simulink subsystem "complementaryFilter"  (R2026a)
settings: Solver=VariableStepAuto
values from neighbouring files (symbols this model uses):
  navComp = 0.995    [navParams.sldd]
  navControl = 1    [navParams.sldd]
undefined symbols (not defined in the file or in its folder): flightMode
libraries: simulink x3, vrlib x1, sharedutil x1
settings Model: Creator=maxhu  LastModifiedBy=maxhu

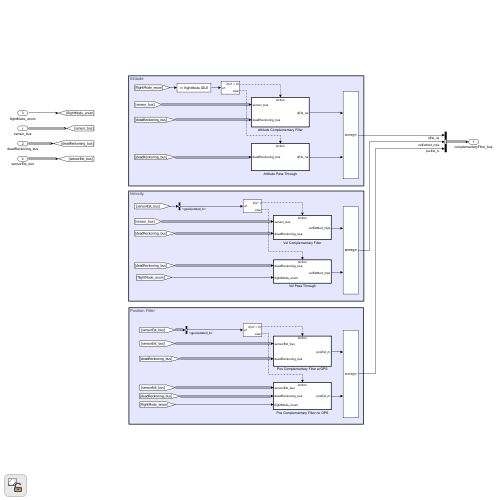
[thumbnail: Simulink's stored preview of the top-level diagram]
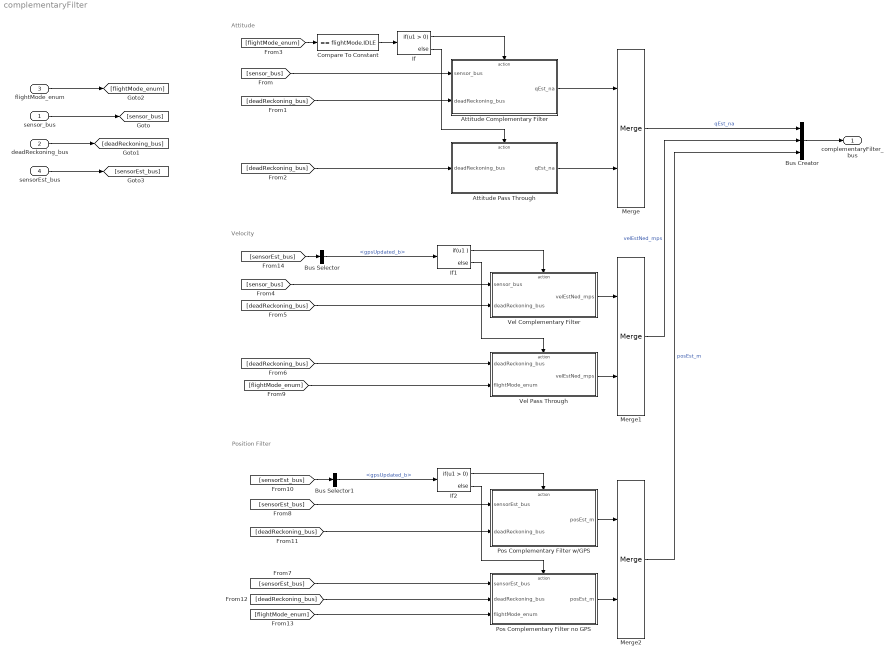
== system complementaryFilter ==
  note: Position Filter
  note: Attitude
  note: Velocity
  sensor_bus : Inport
  deadReckoning_bus : Inport  Port=2
  flightMode_enum : Inport  Port=3
  sensorEst_bus : Inport  Port=4
  Attitude Complementary Filter : Subsystem  TreatAsAtomicUnit=on
  Attitude Pass Through : Subsystem  TreatAsAtomicUnit=on
  Bus Creator : BusCreator  Inputs=3
  Bus Selector : BusSelector  OutputSignals=gpsUpdated_b
  Bus Selector1 : BusSelector  OutputSignals=gpsUpdated_b
  Compare To Constant : simulink/Logic and Bit Operations/Compare To Constant  relop===  const=flightMode.IDLE  OutDataTypeStr=boolean
  If : If
  If1 : If  IfExpression=u1
  If2 : If
  Merge : Merge
  Merge1 : Merge
  Merge2 : Merge
  Pos Complementary Filter no GPS : Subsystem  TreatAsAtomicUnit=on
  Pos Complementary Filter w/GPS : Subsystem  TreatAsAtomicUnit=on
  Vel Complementary Filter : Subsystem  TreatAsAtomicUnit=on
  Vel Pass Through : Subsystem  TreatAsAtomicUnit=on
  complementaryFilter_bus : Outport
  wires:
  Merge/1 -> Bus Creator/1  "qEst_na"
  Bus Creator/1 -> complementaryFilter_bus/1
  Compare To Constant/1 -> If/1
  If/1 -> Attitude Complementary Filter/Action
  If/2 -> Attitude Pass Through/Action
  Attitude Complementary Filter/1(qEst_na) -> Merge/1
  Attitude Pass Through/1(qEst_na) -> Merge/2
  [sensor_bus] -> Attitude Complementary Filter/1(sensor_bus)
  [deadReckoning_bus] -> Attitude Complementary Filter/2(deadReckoning_bus)
  [deadReckoning_bus] -> Attitude Pass Through/1(deadReckoning_bus)
  [flightMode_enum] -> Compare To Constant/1
  sensor_bus/1 -> [sensor_bus]
  deadReckoning_bus/1 -> [deadReckoning_bus]
  flightMode_enum/1 -> [flightMode_enum]
  Merge2/1 -> Bus Creator/3  "posEst_m"
  sensorEst_bus/1 -> [sensorEst_bus]
  If2/2 -> Pos Complementary Filter no GPS/Action
  Pos Complementary Filter no GPS/1(posEst_m) -> Merge2/2
  Pos Complementary Filter w/GPS/1(posEst_m) -> Merge2/1
  Bus Selector1/1 -> If2/1  "<gpsUpdated_b>"
  If2/1 -> Pos Complementary Filter w/GPS/Action
  [deadReckoning_bus] -> Pos Complementary Filter w/GPS/2(deadReckoning_bus)
  [deadReckoning_bus] -> Pos Complementary Filter no GPS/2(deadReckoning_bus)
  [sensorEst_bus] -> Pos Complementary Filter no GPS/1(sensorEst_bus)
  [sensorEst_bus] -> Pos Complementary Filter w/GPS/1(sensorEst_bus)
  [flightMode_enum] -> Pos Complementary Filter no GPS/3(flightMode_enum)
  If1/2 -> Vel Pass Through/Action
  Vel Complementary Filter/1(velEstNed_mps) -> Merge1/1
  [deadReckoning_bus] -> Vel Pass Through/1(deadReckoning_bus)
  Bus Selector/1 -> If1/1  "<gpsUpdated_b>"
  [flightMode_enum] -> Vel Pass Through/2(flightMode_enum)
  If1/1 -> Vel Complementary Filter/Action
  Vel Pass Through/1(velEstNed_mps) -> Merge1/2
  [sensor_bus] -> Vel Complementary Filter/1(sensor_bus)
  [deadReckoning_bus] -> Vel Complementary Filter/2(deadReckoning_bus)
  Merge1/1 -> Bus Creator/2  "velEstNed_mps"
  [sensorEst_bus] -> Bus Selector/1
  [sensorEst_bus] -> Bus Selector1/1

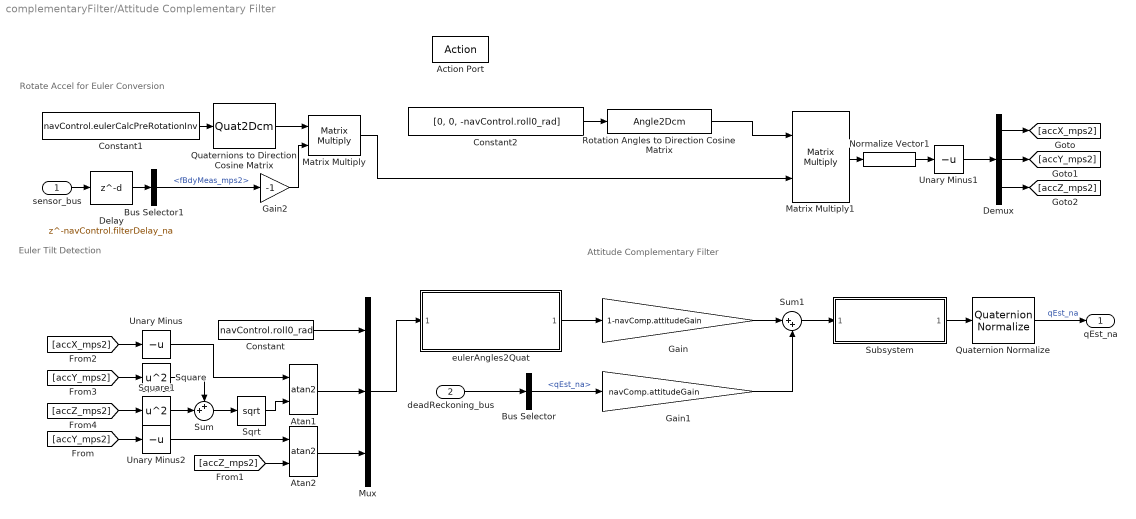
== system complementaryFilter/Attitude Complementary Filter ==
  note: Rotate Accel for Euler Conversion
  note: Euler Tilt Detection
  note: Attitude Complementary Filter
  sensor_bus : Inport
  deadReckoning_bus : Inport  Port=2
  Action Port : ActionPort
  Atan1 : Trigonometry  Operator=atan2
  Atan2 : Trigonometry  Operator=atan2
  Bus Selector : BusSelector  OutputSignals=qEst_na
  Bus Selector1 : BusSelector  OutputSignals=fBdyMeas_mps2
  Constant : Constant  Value=navControl.roll0_rad
  Constant1 : Constant  Value=navControl.eulerCalcPreRotationInv
  Constant2 : Constant  Value=[0, 0, -navControl.roll0_rad]
  Delay : Delay  DelayLength=navControl.filterDelay_na
  Demux : Demux  Outputs=3
  Gain : Gain  Gain=1-navComp.attitudeGain
  Gain1 : Gain  Gain=navComp.attitudeGain
  Gain2 : Gain  Gain=-1
  Matrix Multiply : Product  Multiplication=Matrix(*)
  Matrix Multiply1 : Product  Multiplication=Matrix(*)
  Mux : Mux  Inputs=3
  Normalize Vector1 : vrlib/Utilities/Normalize Vector  maxzero=1e-6
  Quaternion Normalize : sharedutil/Quaternion Normalize  aMode=aMode
  Quaternions to Direction Cosine Matrix : Quat2Dcm
  Rotation Angles to Direction Cosine Matrix : Angle2Dcm  rotationOrder=XYZ
      settings: AttributesFormatString=Rotation Order: %<rotationOrder>
  Sqrt : Sqrt
  Square : Math  Operator=square
  Square1 : Math  Operator=square
  Subsystem : Subsystem  ReferencedSubsystem=removeQuatZero
  Sum : Sum  Inputs=++|
  Sum1 : Sum  Inputs=|++
  Unary Minus : UnaryMinus
  Unary Minus1 : UnaryMinus
  Unary Minus2 : UnaryMinus
  eulerAngles2Quat : Subsystem  ReferencedSubsystem=eulerAngles2Quat
  qEst_na : Outport
  wires:
  Constant2/1 -> Rotation Angles to Direction Cosine Matrix/1
  Rotation Angles to Direction Cosine Matrix/1 -> Matrix Multiply1/1
  Constant/1 -> Mux/1
  Matrix Multiply1/1 -> Normalize Vector1/1
  Matrix Multiply/1 -> Matrix Multiply1/2
  Unary Minus2/1 -> Atan2/1
  Atan2/1 -> Mux/3
  Atan1/1 -> Mux/2
  Unary Minus1/1 -> Demux/1
  Normalize Vector1/1 -> Unary Minus1/1
  Unary Minus/1 -> Atan1/1
  Sqrt/1 -> Atan1/2
  [accY_mps2] -> Unary Minus2/1
  [accZ_mps2] -> Atan2/2
  Gain/1 -> Sum1/1
  [accY_mps2] -> Square/1
  Gain1/1 -> Sum1/2
  Square/1 -> Sum/1
  Sum/1 -> Sqrt/1
  eulerAngles2Quat/1 -> Gain/1
  Demux/1 -> [accX_mps2]
  Square1/1 -> Sum/2
  Demux/2 -> [accY_mps2]
  Demux/3 -> [accZ_mps2]
  [accX_mps2] -> Unary Minus/1
  [accZ_mps2] -> Square1/1
  deadReckoning_bus/1 -> Bus Selector/1
  Bus Selector/1 -> Gain1/1  "<qEst_na>"
  Gain2/1 -> Matrix Multiply/2
  sensor_bus/1 -> Delay/1
  Bus Selector1/1 -> Gain2/1  "<fBdyMeas_mps2>"
  Delay/1 -> Bus Selector1/1
  Quaternions to Direction Cosine Matrix/1 -> Matrix Multiply/1
  Constant1/1 -> Quaternions to Direction Cosine Matrix/1
  Mux/1 -> eulerAngles2Quat/1
  Quaternion Normalize/1 -> qEst_na/1  "qEst_na"
  Subsystem/1 -> Quaternion Normalize/1
  Sum1/1 -> Subsystem/1

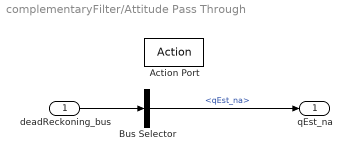
== system complementaryFilter/Attitude Pass Through ==
  deadReckoning_bus : Inport
  Action Port : ActionPort
  Bus Selector : BusSelector  OutputSignals=qEst_na
  qEst_na : Outport
  wires:
  Bus Selector/1 -> qEst_na/1  "<qEst_na>"
  deadReckoning_bus/1 -> Bus Selector/1

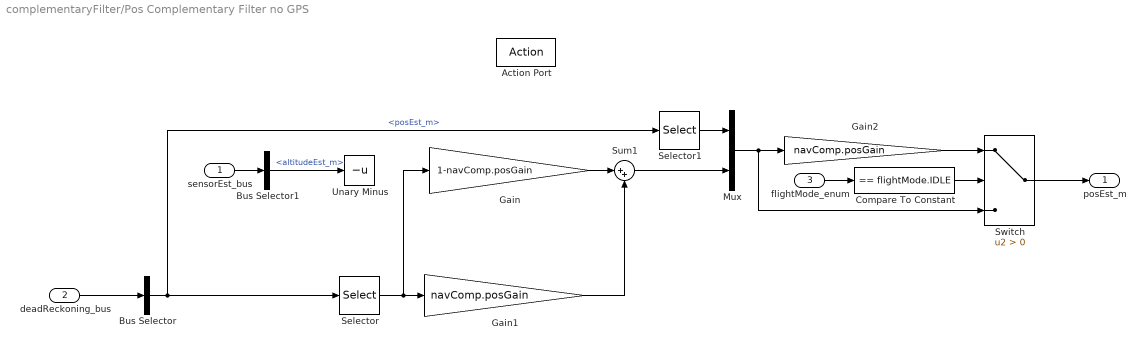
== system complementaryFilter/Pos Complementary Filter no GPS ==
  sensorEst_bus : Inport
  deadReckoning_bus : Inport  Port=2
  flightMode_enum : Inport  Port=3
  Action Port : ActionPort
  Bus Selector : BusSelector  OutputSignals=posEst_m
  Bus Selector1 : BusSelector  OutputSignals=altitudeEst_m
  Compare To Constant : simulink/Logic and Bit Operations/Compare To Constant  relop===  const=flightMode.IDLE  OutDataTypeStr=boolean
  Gain : Gain  Gain=1-navComp.posGain
  Gain1 : Gain  Gain=navComp.posGain
  Gain2 : Gain  Gain=navComp.posGain
  Mux : Mux  Inputs=2
  Selector : Selector  InputPortWidth=3  IndexOptions=Index vector (dialog)  Indices=[3]  OutputSizes=1
  Selector1 : Selector  InputPortWidth=3  IndexOptions=Index vector (dialog)  Indices=[1 2]  OutputSizes=1
  Sum1 : Sum  Inputs=|++
  Switch : Switch  Criteria=u2 > Threshold  SaturateOnIntegerOverflow=off  InputSameDT=off
  Unary Minus : UnaryMinus
  posEst_m : Outport
  wires:
  Mux/1 -> Gain2/1, Switch/3
  flightMode_enum/1 -> Compare To Constant/1
  Gain2/1 -> Switch/1
  Compare To Constant/1 -> Switch/2
  Selector1/1 -> Mux/1
  Sum1/1 -> Mux/2
  Gain/1 -> Sum1/1
  Gain1/1 -> Sum1/2
  Bus Selector1/1 -> Unary Minus/1  "<altitudeEst_m>"
  sensorEst_bus/1 -> Bus Selector1/1
  deadReckoning_bus/1 -> Bus Selector/1
  Bus Selector/1 -> Selector/1, Selector1/1  "<posEst_m>"
  Switch/1 -> posEst_m/1
  Selector/1 -> Gain1/1, Gain/1

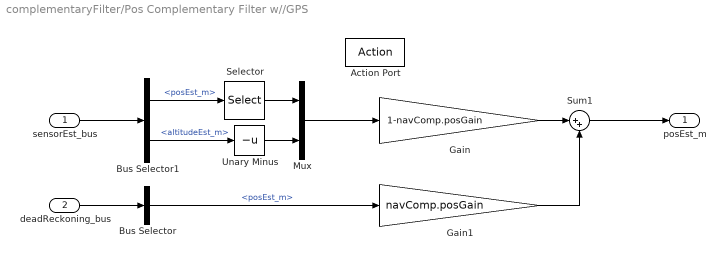
== system complementaryFilter/Pos Complementary Filter w//GPS ==
  sensorEst_bus : Inport
  deadReckoning_bus : Inport  Port=2
  Action Port : ActionPort
  Bus Selector : BusSelector  OutputSignals=posEst_m
  Bus Selector1 : BusSelector  OutputSignals=posEst_m,altitudeEst_m
  Gain : Gain  Gain=1-navComp.posGain
  Gain1 : Gain  Gain=navComp.posGain
  Mux : Mux  Inputs=2
  Selector : Selector  InputPortWidth=3  IndexOptions=Index vector (dialog)  Indices=[1 2]  OutputSizes=1
  Sum1 : Sum  Inputs=|++
  Unary Minus : UnaryMinus
  posEst_m : Outport
  wires:
  Mux/1 -> Gain/1
  Unary Minus/1 -> Mux/2
  Selector/1 -> Mux/1
  Bus Selector1/1 -> Selector/1  "<posEst_m>"
  Bus Selector1/2 -> Unary Minus/1  "<altitudeEst_m>"
  sensorEst_bus/1 -> Bus Selector1/1
  Gain/1 -> Sum1/1
  Gain1/1 -> Sum1/2
  deadReckoning_bus/1 -> Bus Selector/1
  Bus Selector/1 -> Gain1/1  "<posEst_m>"
  Sum1/1 -> posEst_m/1

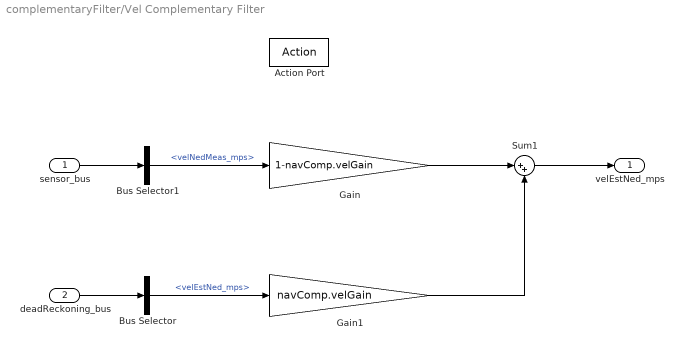
== system complementaryFilter/Vel Complementary Filter ==
  sensor_bus : Inport
  deadReckoning_bus : Inport  Port=2
  Action Port : ActionPort
  Bus Selector : BusSelector  OutputSignals=velEstNed_mps
  Bus Selector1 : BusSelector  OutputSignals=velNedMeas_mps
  Gain : Gain  Gain=1-navComp.velGain
  Gain1 : Gain  Gain=navComp.velGain
  Sum1 : Sum  Inputs=|++
  velEstNed_mps : Outport
  wires:
  Gain/1 -> Sum1/1
  sensor_bus/1 -> Bus Selector1/1
  Gain1/1 -> Sum1/2
  Bus Selector1/1 -> Gain/1  "<velNedMeas_mps>"
  deadReckoning_bus/1 -> Bus Selector/1
  Bus Selector/1 -> Gain1/1  "<velEstNed_mps>"
  Sum1/1 -> velEstNed_mps/1

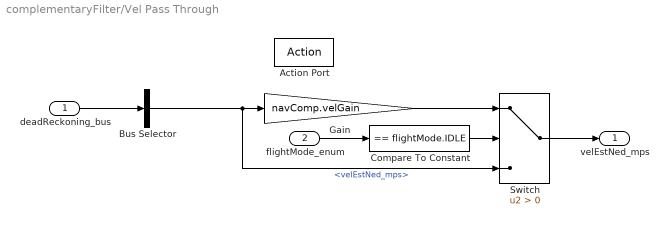
== system complementaryFilter/Vel Pass Through ==
  deadReckoning_bus : Inport
  flightMode_enum : Inport  Port=2
  Action Port : ActionPort
  Bus Selector : BusSelector  OutputSignals=velEstNed_mps
  Compare To Constant : simulink/Logic and Bit Operations/Compare To Constant  relop===  const=flightMode.IDLE  OutDataTypeStr=boolean
  Gain : Gain  Gain=navComp.velGain
  Switch : Switch  Criteria=u2 > Threshold  SaturateOnIntegerOverflow=off  InputSameDT=off
  velEstNed_mps : Outport
  wires:
  Gain/1 -> Switch/1
  Switch/1 -> velEstNed_mps/1
  Bus Selector/1 -> Gain/1, Switch/3  "<velEstNed_mps>"
  Compare To Constant/1 -> Switch/2
  flightMode_enum/1 -> Compare To Constant/1
  deadReckoning_bus/1 -> Bus Selector/1
